simulink subsystem "abc_Limiter"  (R2022b)
settings: Solver=VariableStepAuto  StartTime=0.0  StopTime=10.0  RelTol=1e-3
model mask{max_amplitude=1, T_s_dq=1e-3, T_s_theta=1e-4, datatype='double'}
  mask prompts: T_s_dq "Input vector sample time [s]"; T_s_theta "Angle theta sample time [s]"; datatype "Signal data type"
libraries: eeTransforms x3, simulink x3
settings Model: Creator=winkens  LastModifiedBy=winkens
settings SolverCC: AlgebraicLoopSolver=TrustRegion
settings DebuggingCC: UnconnectedInputMsg=warning  UnconnectedOutputMsg=warning  UnconnectedLineMsg=warning  SFMachineParentedDataDiag=warning
settings ModelReferenceCC: EnableRefExpFcnMdlSchedulingChecks=on
settings RTWCC: DLArmComputeVersion=19.05

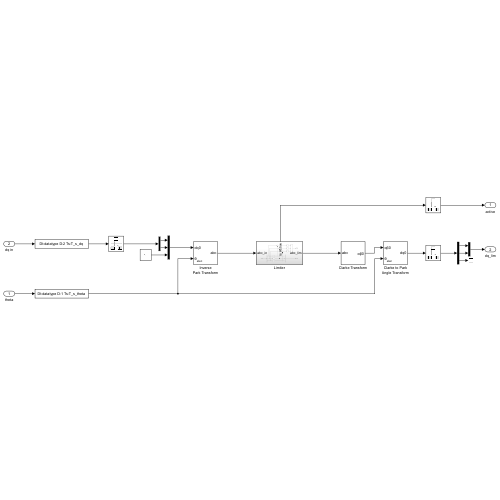
[thumbnail: Simulink's stored preview of the top-level diagram]
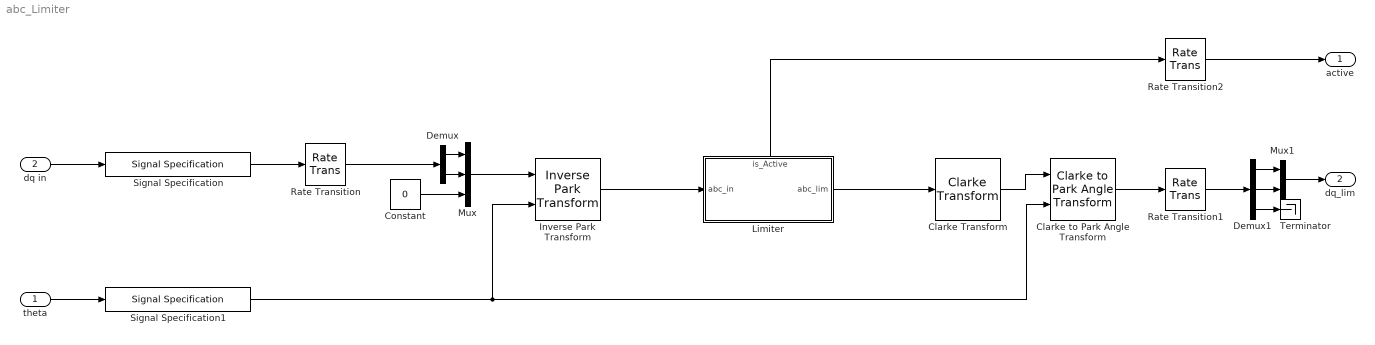
== system abc_Limiter ==
  theta : Inport
  dq in : Inport  Port=2
  Clarke Transform : eeTransforms/Clarke Transform  PowerInvariant=off
  Clarke to Park Angle Transform : eeTransforms/Clarke to Park Angle Transform  AxisAlignment=D-axis
  Constant : Constant  Value=0  OutDataTypeStr=datatype
  Demux : Demux  Outputs=2
  Demux1 : Demux  Outputs=3
  Inverse Park Transform : eeTransforms/Inverse Park Transform  AxisAlignment=D-axis  PowerInvariant=off
  Limiter : Subsystem
      settings: PortSchema="{\"entries\":[{\"content\":{\"sides\":[{\"content\":{\"connectorIds\":[\"In1\"]},\"type\":\"ConnectorPlacement.EquallySpacedRectSide\",\"uuid\":\"f729261e-1035-4e52-9deb-1657aace88d9\"},{\"content\":{\"connectorIds\":[\"Out1\"],\"side\":\"RIGHT\"},\"type\":\"ConnectorPlacement.EquallySpacedRectSide\",\"uuid\":\"97a47801-9405-4c20-848c-4b15225d8d1b\"},{\"content\":{\"connectorIds\":[\"Out2\"],\"side\":\"TOP\"},\"type\":\"ConnectorPlacement.EquallySpacedRectSide\",\"uuid\":\"3dd00258-aa34-4bf8-bfda-f65b16cec211\"}]},\"type\":\"ConnectorPlacement.EquallySpacedConnector\",\"uuid\":\"bb524402-4a0a-4c60-8c37-17c73cb46b69\"}],\"packageUris\":[\"http://schema.mathworks.com/mf0/Connector/R2020b\"],\"version\":\"1.0\"}"
  Mux : Mux  Inputs=3
  Mux1 : Mux  Inputs=2
  Rate Transition : RateTransition  Deterministic=off  OutPortSampleTime=T_s_theta
  Rate Transition1 : RateTransition  Deterministic=off  OutPortSampleTime=T_s_dq
  Rate Transition2 : RateTransition  Deterministic=off  OutPortSampleTime=T_s_dq
  Signal Specification : SignalSpecification  OutDataTypeStr=datatype  Dimensions=2  SampleTime=T_s_dq
  Signal Specification1 : SignalSpecification  OutDataTypeStr=datatype  Dimensions=1  SampleTime=T_s_theta
  Terminator : Terminator
  active : Outport
  dq_lim : Outport  Port=2
  wires:
  dq in/1 -> Signal Specification/1
  Mux1/1 -> dq_lim/1
  Rate Transition2/1 -> active/1
  Demux/1 -> Mux/1
  Demux/2 -> Mux/2
  Constant/1 -> Mux/3
  Mux/1 -> Inverse Park Transform/1
  theta/1 -> Signal Specification1/1
  Clarke Transform/1 -> Clarke to Park Angle Transform/1
  Demux1/1 -> Mux1/1
  Demux1/2 -> Mux1/2
  Clarke to Park Angle Transform/1 -> Rate Transition1/1
  Demux1/3 -> Terminator/1
  Rate Transition/1 -> Demux/1
  Rate Transition1/1 -> Demux1/1
  Signal Specification/1 -> Rate Transition/1
  Signal Specification1/1 -> Clarke to Park Angle Transform/2, Inverse Park Transform/2
  Inverse Park Transform/1 -> Limiter/1(abc_in)
  Limiter/1(abc_lim) -> Clarke Transform/1
  Limiter/2(is_Active) -> Rate Transition2/1

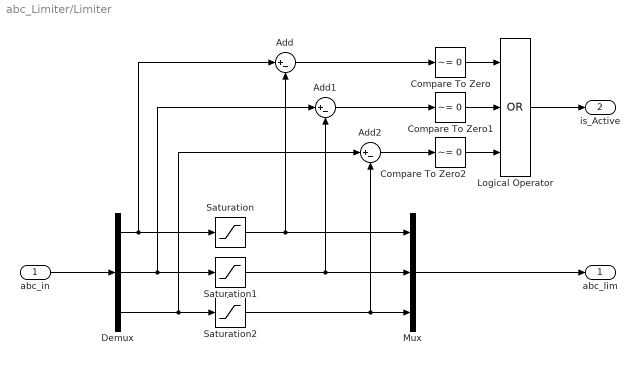
== system abc_Limiter/Limiter ==
  abc_in : Inport
  Add : Sum  Inputs=|+-
  Add1 : Sum  Inputs=|+-
  Add2 : Sum  Inputs=|+-
  Compare To Zero : simulink/Logic and Bit Operations/Compare To Zero  relop=~=  OutDataTypeStr=boolean
  Compare To Zero1 : simulink/Logic and Bit Operations/Compare To Zero  relop=~=  OutDataTypeStr=boolean
  Compare To Zero2 : simulink/Logic and Bit Operations/Compare To Zero  relop=~=  OutDataTypeStr=boolean
  Demux : Demux  Outputs=3
  Logical Operator : Logic  Operator=OR  Inputs=3  AllPortsSameDT=off  OutDataTypeStr=boolean
  Mux : Mux  Inputs=3
  Saturation : Saturate  UpperLimit=max_amplitude  LowerLimit=- max_amplitude
  Saturation1 : Saturate  UpperLimit=max_amplitude  LowerLimit=- max_amplitude
  Saturation2 : Saturate  UpperLimit=max_amplitude  LowerLimit=- max_amplitude
  abc_lim : Outport
  is_Active : Outport  Port=2
  wires:
  abc_in/1 -> Demux/1
  Demux/1 -> Add/1, Saturation/1
  Demux/2 -> Add1/1, Saturation1/1
  Demux/3 -> Add2/1, Saturation2/1
  Saturation/1 -> Add/2, Mux/1
  Saturation1/1 -> Add1/2, Mux/2
  Saturation2/1 -> Add2/2, Mux/3
  Mux/1 -> abc_lim/1
  Add2/1 -> Compare To Zero2/1
  Add1/1 -> Compare To Zero1/1
  Add/1 -> Compare To Zero/1
  Compare To Zero/1 -> Logical Operator/1
  Compare To Zero1/1 -> Logical Operator/2
  Compare To Zero2/1 -> Logical Operator/3
  Logical Operator/1 -> is_Active/1
